simulink model "chaine_base"  (R2023b)
settings: Solver=FixedStepDiscrete  StartTime=0.0  StopTime=10000  FixedStep=Te  RelTol=1e-3
values from neighbouring files (symbols this model uses):
  A = P.A    [P3_Q10_parametres_integration.m]    (also in P3_Q11_variance_integrateur.m; P3_Q12_TEB.m; P3_Q4_bruit_uniforme.m; P3_Q5_erreur_uniforme.m)
  L = P.L    [P3_Q10_parametres_integration.m]    (also in P3_Q11_variance_integrateur.m; P3_Q12_TEB.m; P3_Q13_integration.m; P3_parametres.m)
  P = parametres_perso('LABBE Emmy')    [P2_Q11_LZ78_convergence.m]    (also in P2_Q1_source_binaire_simulation.m; P2_Q7_extension_source.m; P3_Q10_parametres_integration.m; P3_Q11_variance_integrateur.m)
  sigma2_bruit = N0 * L / (2*Tb)    [P3_Q10_parametres_integration.m]    (also in P3_parametres.m)
  Tb = 1;')    [LANCER_TP_COMPLET.m]    (also in P2_Q1_source_binaire_simulation.m = 1; P3_Q10_parametres_integration.m = 1; P3_Q11_variance_integrateur.m = 1; P3_Q12_TEB.m = 1)
  Te = Tb / L    [P3_Q10_parametres_integration.m]    (also in P3_Q11_variance_integrateur.m; P3_Q12_TEB.m; P3_parametres.m = Tb/L)
libraries: simulink x2, dspstat3 x1
settings Model: Creator=e2202522  LastModifiedBy=e2202522

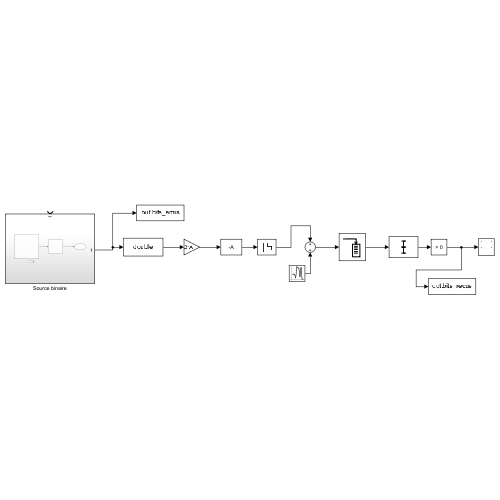
[thumbnail: Simulink's stored preview of the top-level diagram]
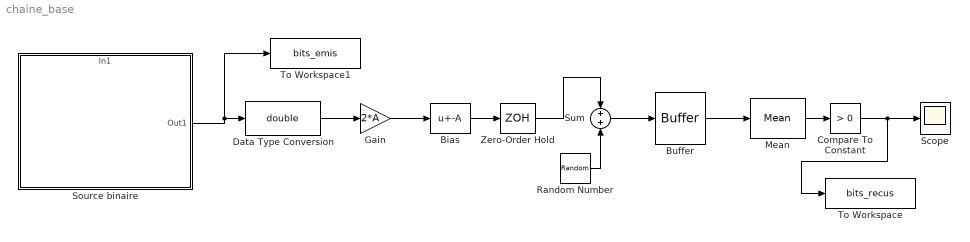
== system chaine_base ==
  Bias : Bias  Bias=-A  SaturateOnIntegerOverflow=off
  Buffer : Buffer  N=L  OutputFrames=off
  Compare To Constant : simulink/Logic and Bit Operations/Compare To Constant  relop=>  const=0  OutDataTypeStr=boolean
  Data Type Conversion : DataTypeConversion  OutDataTypeStr=double  SaturateOnIntegerOverflow=off  RndMeth=Floor
  Gain : Gain  Gain=2*A
  Mean : dspstat3/Mean  run=off  InputProcessing=Columns as channels (frame based)  reset_popup=None  directionMode=Each column  dimension=1  roiEnable=off  roiType=Rectangles  roiPortion=Entire ROI  roiOutput=Individual statistics for each ROI  roiFlag=off  roundingMode=Floor  overflowMode=off  outputDataTypeStr=Inherit: Same as accumulator  outputMin=[]  outputMax=[]  outputLastDataTypeStr=Inherit: Same as accumulator
  Random Number : RandomNumber  Variance=sigma2_bruit  Seed=P.graine  SampleTime=Te
  Scope : Scope
  Source binaire : Subsystem
      settings: PortSchema="{\"entries\":[{\"content\":{\"sides\":[{\"content\":{},\"type\":\"ConnectorPlacement.EquallySpacedRectSide\",\"uuid\":\"1d1b3a40-eee1-4311-a28c-a5c990f69d61\"},{\"content\":{\"connectorIds\":[\"Out1\"],\"side\":\"RIGHT\"},\"type\":\"ConnectorPlacement.EquallySpacedRectSide\",\"uuid\":\"9115f35c-513c-4ea1-a40d-1e1aebcfde17\"},{\"content\":{\"connectorIds\":[\"In1\"],\"side\":\"TOP\"},\"type\":\"ConnectorPlacement.EquallySpacedRectSide\",\"uuid\":\"a6426102-e6a6-474b-a4e7-9dc638e2ca24\"}]},\"type\":\"ConnectorPlacement.EquallySpacedConnector\",\"uuid\":\"766fcb99-2af9-4dfe-9edb-f04684085cad\"}],\"packageUris\":[\"http://schema.mathworks.com/mf0/Connector/R2020b\"],\"version\":\"1.0\"}"
  Sum : Sum
  To Workspace : ToWorkspace  VariableName=bits_recus  SampleTime=-1
  To Workspace1 : ToWorkspace  VariableName=bits_emis  SampleTime=-1
  Zero-Order Hold : ZeroOrderHold  SampleTime=Te
  wires:
  Source binaire/1(Out1) -> To Workspace1/1, Data Type Conversion/1
  Data Type Conversion/1 -> Gain/1
  Gain/1 -> Bias/1
  Bias/1 -> Zero-Order Hold/1
  Zero-Order Hold/1 -> Sum/1
  Random Number/1 -> Sum/2
  Sum/1 -> Buffer/1
  Buffer/1 -> Mean/1
  Mean/1 -> Compare To Constant/1
  Compare To Constant/1 -> To Workspace/1, Scope/1

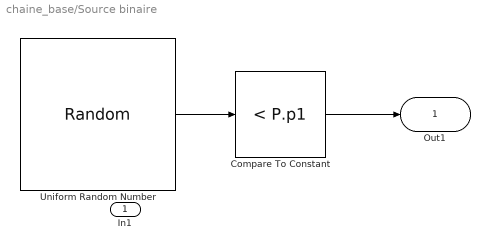
== system chaine_base/Source binaire ==
  In1 : Inport
  Compare To Constant : simulink/Logic and Bit Operations/Compare To Constant  relop=<  const=P.p1  OutDataTypeStr=boolean
  Uniform Random Number : UniformRandomNumber  Minimum=0  Seed=P.graine  SampleTime=Tb
  Out1 : Outport
  wires:
  Compare To Constant/1 -> Out1/1
  Uniform Random Number/1 -> Compare To Constant/1
